simulink model "Controller"  (R2018b)
settings: configuration reference "control_config" (kept outside this file)
values from neighbouring files (symbols this model uses):
  CONTROL_EXPORT = Simulink.Parameter(CONTROL_EXPORT_VALUE)    [controller_model_init.m]
  CONTROL_PARAM = Simulink.Parameter(CONTROL_PARAM_VALUE)    [controller_model_init.m]
undefined symbols (not defined in the file or in its folder): actuator_cmd, CONTROL_CONST, DiscIntNeverNeededParam, timestamp
libraries: FMT_Model_Lib x5, simulink x1
settings Model: Creator=jc  LastModifiedBy=zouji
settings ConfigSetRef: SourceLocation=Base Workspace

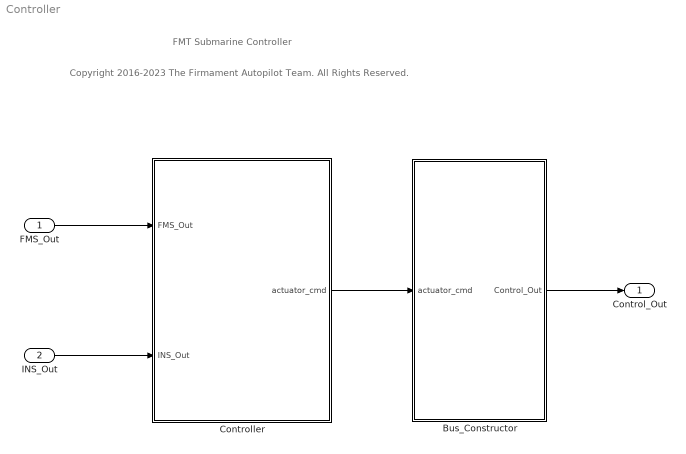
== system Controller ==
  note: Copyright 2016-2023 The Firmament Autopilot Team. All Rights Reserved.
  note: FMT Submarine Controller
  FMS_Out : Inport  OutDataTypeStr=Bus: FMS_Out_Bus
  INS_Out : Inport  Port=2  OutDataTypeStr=Bus: INS_Out_Bus
  Bus_Constructor : Subsystem
  Controller : Subsystem
  Control_Out : Outport  OutDataTypeStr=Bus: Control_Out_Bus
  wires:
  FMS_Out/1 -> Controller/1(FMS_Out)
  INS_Out/1 -> Controller/2(INS_Out)
  Controller/1(actuator_cmd) -> Bus_Constructor/1(actuator_cmd)
  Bus_Constructor/1(Control_Out) -> Control_Out/1

== system Controller/Bus_Constructor ==
  actuator_cmd : Inport
  Bus Assignment : BusAssignment  AssignedSignals=actuator_cmd,timestamp
  Constant : Constant  Value=0  OutDataTypeStr=Bus: Control_Out_Bus
  timestamp : Subsystem  mask{sample_time=CONTROL_EXPORT.period}
      mask prompts: sample_time "sample time (ms)"
  Control_Out : Outport
  wires:
  actuator_cmd/1 -> Bus Assignment/2
  Constant/1 -> Bus Assignment/1
  Bus Assignment/1 -> Control_Out/1
  timestamp/1(timestamp_ms) -> Bus Assignment/3

== system Controller/Controller ==
  FMS_Out : Inport
  INS_Out : Inport  Port=2
  Attitude_Controller : Subsystem
  Control_Allocation : Subsystem  Variant=on
      settings: GeneratePreprocessorConditionals=on
  Velocity_Controller : Subsystem
  actuator_cmd : Outport
  wires:
  Control_Allocation/1(actuator_cmd) -> actuator_cmd/1
  Attitude_Controller/1(torque_cmd_B) -> Control_Allocation/2(ang_acc_cmd)
  Velocity_Controller/1(force_cmd_B) -> Control_Allocation/3(line_acc_cmd)
  FMS_Out/1 -> Velocity_Controller/1(FMS_Out), Control_Allocation/1(FMS_Out), Attitude_Controller/1(FMS_Out)
  INS_Out/1 -> Velocity_Controller/2(INS_Out), Attitude_Controller/2(INS_Out)

== system Controller/Bus_Constructor/timestamp ==
  Constant : Constant  Value=sample_time
  Data Type Conversion : DataTypeConversion  OutDataTypeStr=uint32
  Discrete-Time Integrator : DiscreteIntegrator  IntegratorMethod=Accumulation: Forward Euler  SampleTime=-1  ICPrevOutput=DiscIntNeverNeededParam  ICPrevScaledInput=DiscIntNeverNeededParam
  timestamp_ms : Outport
  wires:
  Discrete-Time Integrator/1 -> Data Type Conversion/1
  Constant/1 -> Discrete-Time Integrator/1
  Data Type Conversion/1 -> timestamp_ms/1

== system Controller/Controller/Attitude_Controller ==
  FMS_Out : Inport
  INS_Out : Inport  Port=2
  Inner_Loop : Subsystem
  Outter_Loop : Subsystem
  Saturation1 : Saturate  UpperLimit=1  LowerLimit=-1
  torque_cmd_B : Outport
  wires:
  INS_Out/1 -> Inner_Loop/2(INS_Out), Outter_Loop/1(INS_Out)
  FMS_Out/1 -> Inner_Loop/3(FMS_Out), Outter_Loop/2(FMS_Out)
  Outter_Loop/1(rate_cmd_radPs) -> Inner_Loop/1(rate_cmd_radPs)
  Inner_Loop/1(rate_dot_cmd_B) -> Saturation1/1
  Saturation1/1 -> torque_cmd_B/1

== system Controller/Controller/Control_Allocation ==
  note: 1) Add Subsystem or Model blocks as valid variant choices.
      | 2) You cannot connect blocks at this level. At simulation, connectivity is automatically
      | determined, based on the active variant and port name matching.
  FMS_Out : Inport
  ang_acc_cmd : Inport  Port=2
  line_acc_cmd : Inport  Port=3
  Submarine_1 : Subsystem  TreatAsAtomicUnit=on  VariantControl=AIRFRAME==1
      mask Display: image('D:\ws\FMT\FMT-Model\figures\submarine_1.png');
  actuator_cmd : Outport

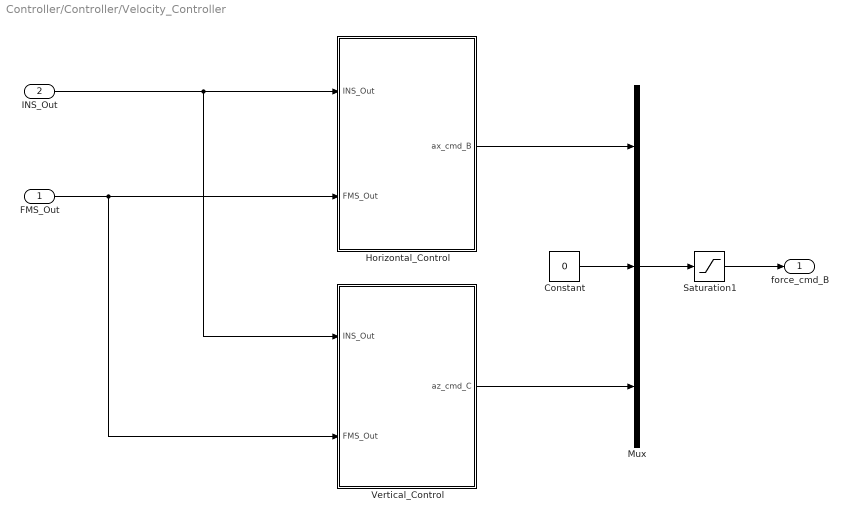
== system Controller/Controller/Velocity_Controller ==
  FMS_Out : Inport
  INS_Out : Inport  Port=2
  Constant : Constant  Value=0  OutDataTypeStr=single
  Horizontal_Control : Subsystem
  Mux : Mux  Inputs=3
  Saturation1 : Saturate  UpperLimit=1  LowerLimit=-1
  Vertical_Control : Subsystem
  force_cmd_B : Outport
  wires:
  FMS_Out/1 -> Vertical_Control/2(FMS_Out), Horizontal_Control/2(FMS_Out)
  Mux/1 -> Saturation1/1
  INS_Out/1 -> Vertical_Control/1(INS_Out), Horizontal_Control/1(INS_Out)
  Horizontal_Control/1(ax_cmd_B) -> Mux/1
  Vertical_Control/1(az_cmd_C) -> Mux/3
  Constant/1 -> Mux/2
  Saturation1/1 -> force_cmd_B/1

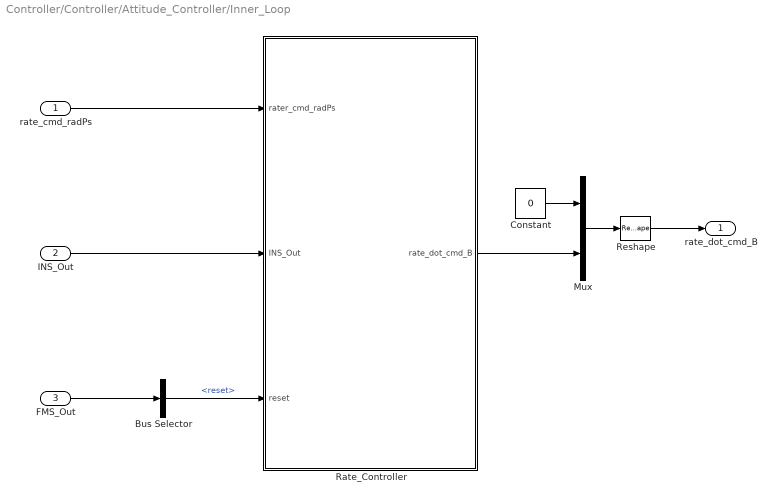
== system Controller/Controller/Attitude_Controller/Inner_Loop ==
  rate_cmd_radPs : Inport
  INS_Out : Inport  Port=2
  FMS_Out : Inport  Port=3
  Bus Selector : BusSelector  OutputSignals=reset
  Constant : Constant  Value=0  OutDataTypeStr=single
  Mux : Mux  Inputs=2
  Rate_Controller : Subsystem
  Reshape : Reshape  OutputDimensionality=Column vector (2-D)
  rate_dot_cmd_B : Outport
  wires:
  Rate_Controller/1(rate_dot_cmd_B) -> Mux/2
  Bus Selector/1 -> Rate_Controller/3(reset)  "<reset>"
  INS_Out/1 -> Rate_Controller/2(INS_Out)
  FMS_Out/1 -> Bus Selector/1
  Mux/1 -> Reshape/1
  Constant/1 -> Mux/1
  rate_cmd_radPs/1 -> Rate_Controller/1(rater_cmd_radPs)
  Reshape/1 -> rate_dot_cmd_B/1

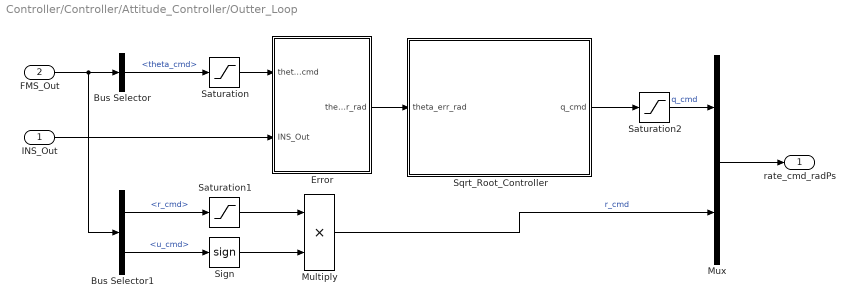
== system Controller/Controller/Attitude_Controller/Outter_Loop ==
  INS_Out : Inport
  FMS_Out : Inport  Port=2
  Bus Selector : BusSelector  OutputSignals=theta_cmd
  Bus Selector1 : BusSelector  OutputSignals=r_cmd,u_cmd
  Error : Subsystem
  Multiply : Product
  Mux : Mux  Inputs=2
  Saturation : Saturate  UpperLimit=CONTROL_PARAM.PITCH_CMD_LIM  LowerLimit=-CONTROL_PARAM.PITCH_CMD_LIM
  Saturation1 : Saturate  UpperLimit=CONTROL_PARAM.R_CMD_LIM  LowerLimit=-CONTROL_PARAM.R_CMD_LIM
  Saturation2 : Saturate  UpperLimit=CONTROL_PARAM.Q_CMD_LIM  LowerLimit=-CONTROL_PARAM.Q_CMD_LIM
  Sign : Signum
  Sqrt_Root_Controller : Subsystem
  rate_cmd_radPs : Outport
  wires:
  Bus Selector/1 -> Saturation/1  "<theta_cmd>"
  FMS_Out/1 -> Bus Selector1/1, Bus Selector/1
  Sqrt_Root_Controller/1(q_cmd) -> Saturation2/1
  Error/1(theta_err_rad) -> Sqrt_Root_Controller/1(theta_err_rad)
  INS_Out/1 -> Error/2(INS_Out)
  Saturation/1 -> Error/1(theta_cmd)
  Bus Selector1/1 -> Saturation1/1  "<r_cmd>"
  Mux/1 -> rate_cmd_radPs/1
  Saturation2/1 -> Mux/1  "q_cmd"
  Bus Selector1/2 -> Sign/1  "<u_cmd>"
  Saturation1/1 -> Multiply/1
  Sign/1 -> Multiply/2
  Multiply/1 -> Mux/2  "r_cmd"

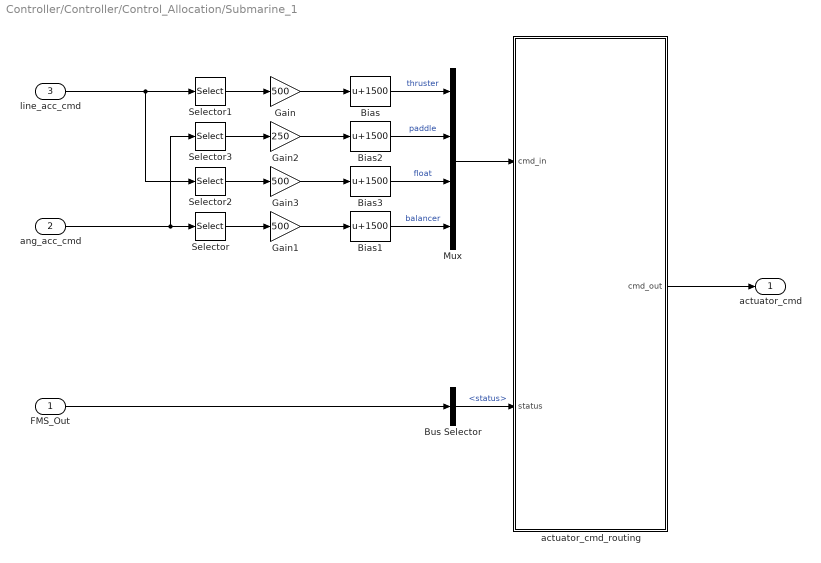
== system Controller/Controller/Control_Allocation/Submarine_1 ==
  FMS_Out : Inport
  ang_acc_cmd : Inport  Port=2
  line_acc_cmd : Inport  Port=3
  Bias{,1..3} (4 alike) : Bias  Bias=1500
  Bus Selector : BusSelector  OutputSignals=status
  Gain : Gain  Gain=500  OutDataTypeStr=uint16
  Gain1 : Gain  Gain=500  OutDataTypeStr=uint16
  Gain2 : Gain  Gain=250  OutDataTypeStr=uint16
  Gain3 : Gain  Gain=500  OutDataTypeStr=uint16
  Mux : Mux
  Selector : Selector  InputPortWidth=3  IndexOptions=Index vector (dialog)  Indices=2  OutputSizes=1
  Selector1 : Selector  InputPortWidth=3  IndexOptions=Index vector (dialog)  Indices=1  OutputSizes=1
  Selector2 : Selector  InputPortWidth=3  IndexOptions=Index vector (dialog)  Indices=3  OutputSizes=1
  Selector3 : Selector  InputPortWidth=3  IndexOptions=Index vector (dialog)  Indices=3  OutputSizes=1
  actuator_cmd_routing : Subsystem
  actuator_cmd : Outport
  wires:
  FMS_Out/1 -> Bus Selector/1
  actuator_cmd_routing/1(cmd_out) -> actuator_cmd/1
  Mux/1 -> actuator_cmd_routing/1(cmd_in)
  Bus Selector/1 -> actuator_cmd_routing/2(status)  "<status>"
  Gain/1 -> Bias/1
  Gain1/1 -> Bias1/1
  ang_acc_cmd/1 -> Selector3/1, Selector/1
  Bias/1 -> Mux/1  "thruster"
  Bias1/1 -> Mux/4  "balancer"
  Gain2/1 -> Bias2/1
  Gain3/1 -> Bias3/1
  Selector1/1 -> Gain/1
  Selector3/1 -> Gain2/1
  Selector2/1 -> Gain3/1
  Bias2/1 -> Mux/2  "paddle"
  Bias3/1 -> Mux/3  "float"
  Selector/1 -> Gain1/1
  line_acc_cmd/1 -> Selector1/1, Selector2/1

== system Controller/Controller/Velocity_Controller/Horizontal_Control ==
  INS_Out : Inport
  FMS_Out : Inport  Port=2
  Bus Selector : BusSelector  OutputSignals=reset
  Error : Subsystem
  PID_Controller : Subsystem
  ax_cmd_B : Outport
  wires:
  Error/1(u_err_B_mPs) -> PID_Controller/1(u_err_B_mPs)
  Bus Selector/1 -> PID_Controller/2(reset)  "<reset>"
  FMS_Out/1 -> Error/2(FMS_Out), Bus Selector/1
  PID_Controller/1(ax_cmd_B) -> ax_cmd_B/1
  INS_Out/1 -> Error/1(INS_Out)

== system Controller/Controller/Velocity_Controller/Vertical_Control ==
  INS_Out : Inport
  FMS_Out : Inport  Port=2
  Bus Selector : BusSelector  OutputSignals=reset
  Error : Subsystem
  PID_Controller : Subsystem
  az_cmd_C : Outport
  wires:
  PID_Controller/1(az_cmd) -> az_cmd_C/1
  Bus Selector/1 -> PID_Controller/2(reset)  "<reset>"
  Error/1(w_cmd_C_mPs) -> PID_Controller/1(w_cmd_C_mPs)
  INS_Out/1 -> Error/2(INS_Out)
  FMS_Out/1 -> Bus Selector/1, Error/1(FMS_Out)

== system Controller/Controller/Attitude_Controller/Inner_Loop/Rate_Controller ==
  rater_cmd_radPs : Inport
  INS_Out : Inport  Port=2
  reset : Inport  Port=3
  Error : Subsystem
  PID_Controller : Subsystem
  rate_dot_cmd_B : Outport
  wires:
  INS_Out/1 -> Error/2(INS_Out)
  Error/1(rate_err_radPs) -> PID_Controller/1(rate_err_C_mPs)
  rater_cmd_radPs/1 -> Error/1(rater_cmd_radPs)
  reset/1 -> PID_Controller/2(reset)
  PID_Controller/1(rate_dot_cmd_C) -> rate_dot_cmd_B/1

== system Controller/Controller/Attitude_Controller/Outter_Loop/Error ==
  theta_cmd : Inport
  INS_Out : Inport  Port=2
  Bus_Select : Subsystem
  Sum : Sum  Inputs=|+-
  theta_err_rad : Outport
  wires:
  theta_cmd/1 -> Sum/1  "theta_cmd_B_rad"
  Sum/1 -> theta_err_rad/1  "theta_error_B_rad"
  INS_Out/1 -> Bus_Select/1(INS_Out)
  Bus_Select/1(theta_est_B_rad) -> Sum/2  "theta_est_B_rad"

== system Controller/Controller/Attitude_Controller/Outter_Loop/Sqrt_Root_Controller ==
  theta_err_rad : Inport
  Constant2 : Constant  Value=CONTROL_PARAM.PITCH_P
  Sqrt_Root_Control : Subsystem  mask{dt=CONTROL_CONST.dt, second_ord_lim=9.5993}
      mask prompts: second_ord_lim "2nd-order lim"
  q_cmd : Outport
  wires:
  Sqrt_Root_Control/1(out) -> q_cmd/1
  theta_err_rad/1 -> Sqrt_Root_Control/1(error)
  Constant2/1 -> Sqrt_Root_Control/2(p)

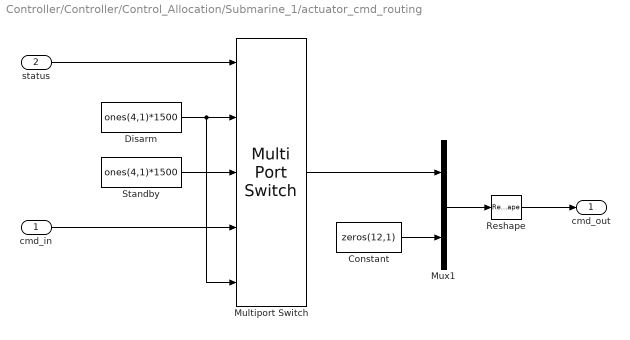
== system Controller/Controller/Control_Allocation/Submarine_1/actuator_cmd_routing ==
  cmd_in : Inport
  status : Inport  Port=2
  Constant : Constant  Value=zeros(12,1)  VectorParams1D=off  OutDataTypeStr=uint16
  Disarm : Constant  Value=ones(4,1)*1500  VectorParams1D=off  OutDataTypeStr=uint16
  Multiport Switch : MultiPortSwitch  DataPortForDefault=Additional data port  DiagnosticForDefault=None
  Mux1 : Mux  Inputs=2
  Reshape : Reshape  OutputDimensionality=Customize  OutputDimensions=[16,1]
  Standby : Constant  Value=ones(4,1)*1500  VectorParams1D=off  OutDataTypeStr=uint16
  cmd_out : Outport
  wires:
  Disarm/1 -> Multiport Switch/5, Multiport Switch/2
  Reshape/1 -> cmd_out/1
  Constant/1 -> Mux1/2
  Standby/1 -> Multiport Switch/3
  Mux1/1 -> Reshape/1
  status/1 -> Multiport Switch/1
  Multiport Switch/1 -> Mux1/1
  cmd_in/1 -> Multiport Switch/4

== system Controller/Controller/Velocity_Controller/Horizontal_Control/Error ==
  INS_Out : Inport
  FMS_Out : Inport  Port=2
  Bus Selector : BusSelector  OutputSignals=u_cmd
  Bus_Select : Subsystem
  Sum : Sum  Inputs=|+-
  u_err_B_mPs : Outport
  wires:
  Sum/1 -> u_err_B_mPs/1  "u_error_B_mPs"
  FMS_Out/1 -> Bus Selector/1
  INS_Out/1 -> Bus_Select/1(INS_Out)
  Bus_Select/1(u_est_B_mPs) -> Sum/2  "u_est_B_mPs"
  Bus Selector/1 -> Sum/1  "<u_cmd>"

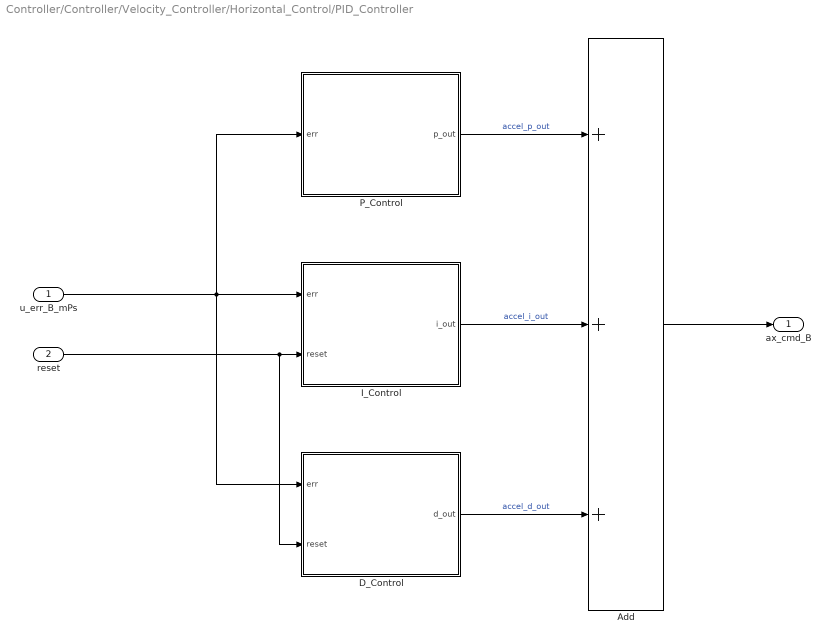
== system Controller/Controller/Velocity_Controller/Horizontal_Control/PID_Controller ==
  u_err_B_mPs : Inport
  reset : Inport  Port=2
  Add : Sum  Inputs=+++
  D_Control : Subsystem  mask{kd=CONTROL_PARAM.VEL_X_D, max_d=CONTROL_PARAM.VEL_X_D_MAX, min_d=CONTROL_PARAM.VEL_X_D_MIN}
  I_Control : Subsystem  mask{ki=CONTROL_PARAM.VEL_X_I, max_i=CONTROL_PARAM.VEL_X_I_MAX, min_i=CONTROL_PARAM.VEL_X_I_MIN}
  P_Control : Subsystem  mask{kp=CONTROL_PARAM.VEL_X_P}
  ax_cmd_B : Outport
  wires:
  u_err_B_mPs/1 -> P_Control/1(err), I_Control/1(err), D_Control/1(err)
  reset/1 -> I_Control/2(reset), D_Control/2(reset)
  P_Control/1(p_out) -> Add/1  "accel_p_out"
  I_Control/1(i_out) -> Add/2  "accel_i_out"
  D_Control/1(d_out) -> Add/3  "accel_d_out"
  Add/1 -> ax_cmd_B/1

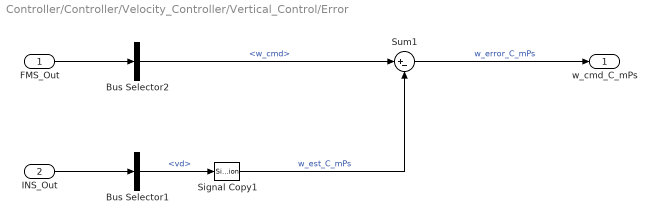
== system Controller/Controller/Velocity_Controller/Vertical_Control/Error ==
  FMS_Out : Inport
  INS_Out : Inport  Port=2
  Bus Selector1 : BusSelector  OutputSignals=vd
  Bus Selector2 : BusSelector  OutputSignals=w_cmd
  Signal Copy1 : SignalConversion  OverrideOpt=off
  Sum1 : Sum  Inputs=|+-
  w_cmd_C_mPs : Outport
  wires:
  INS_Out/1 -> Bus Selector1/1
  Bus Selector2/1 -> Sum1/1  "<w_cmd>"
  Bus Selector1/1 -> Signal Copy1/1  "<vd>"
  Sum1/1 -> w_cmd_C_mPs/1  "w_error_C_mPs"
  FMS_Out/1 -> Bus Selector2/1
  Signal Copy1/1 -> Sum1/2  "w_est_C_mPs"

== system Controller/Controller/Velocity_Controller/Vertical_Control/PID_Controller ==
  w_cmd_C_mPs : Inport
  reset : Inport  Port=2
  Add : Sum  Inputs=+++
  D_Control : Subsystem  mask{kd=CONTROL_PARAM.VEL_Z_D, max_d=CONTROL_PARAM.VEL_Z_D_MAX, min_d=CONTROL_PARAM.VEL_Z_D_MIN}
  I_Control : Subsystem  mask{ki=CONTROL_PARAM.VEL_Z_I, max_i=CONTROL_PARAM.VEL_Z_I_MAX, min_i=CONTROL_PARAM.VEL_Z_I_MIN}
  P_Control : Subsystem  mask{kp=CONTROL_PARAM.VEL_Z_P}
  az_cmd : Outport
  wires:
  P_Control/1(p_out) -> Add/1  "thrust_p_out"
  I_Control/1(i_out) -> Add/2  "thrust_i_out"
  Add/1 -> az_cmd/1
  w_cmd_C_mPs/1 -> D_Control/1(err), I_Control/1(err), P_Control/1(err)
  D_Control/1(d_out) -> Add/3  "thrust_d_out"
  reset/1 -> I_Control/2(reset), D_Control/2(reset)

== system Controller/Controller/Attitude_Controller/Inner_Loop/Rate_Controller/Error ==
  rater_cmd_radPs : Inport
  INS_Out : Inport  Port=2
  Bus_Select : Subsystem
  First Order LPF : FMT_Model_Lib/Filter/First Order LPF  fc=30
      settings: SourceProductName=FMT Toolbox
  Sum : Sum  Inputs=|+-
  rate_err_radPs : Outport
  wires:
  Sum/1 -> First Order LPF/1  "rate_error_B_radPs"
  rater_cmd_radPs/1 -> Sum/1  "rate_cmd_B_radPs"
  INS_Out/1 -> Bus_Select/1(INS_Out)
  Bus_Select/1(rate_est_radPs) -> Sum/2  "rate_est_B_radPs"
  First Order LPF/1 -> rate_err_radPs/1

== system Controller/Controller/Attitude_Controller/Inner_Loop/Rate_Controller/PID_Controller ==
  rate_err_C_mPs : Inport
  reset : Inport  Port=2
  Add : Sum  Inputs=+++
  D_Control : Subsystem  mask{q_kd=CONTROL_PARAM.PITCH_RATE_D, r_kd=CONTROL_PARAM.YAW_RATE_D, max_d=CONTROL_PARAM.RATE_D_MAX, min_d=CONTROL_PARAM.RATE_D_MIN}
  I_Control : Subsystem  mask{q_ki=CONTROL_PARAM.PITCH_RATE_I, r_ki=CONTROL_PARAM.YAW_RATE_I, max_i=CONTROL_PARAM.RATE_I_MAX, min_i=CONTROL_PARAM.RATE_I_MIN}
  P_Control : Subsystem  mask{q_kp=CONTROL_PARAM.PITCH_RATE_P, r_kp=CONTROL_PARAM.YAW_RATE_P}
  rate_dot_cmd_C : Outport
  wires:
  rate_err_C_mPs/1 -> P_Control/1(err), I_Control/1(err), D_Control/1(err)
  reset/1 -> I_Control/2(reset), D_Control/2(reset)
  P_Control/1(p_out) -> Add/1  "accel_p_out"
  I_Control/1(i_out) -> Add/2  "accel_i_out"
  D_Control/1(d_out) -> Add/3  "accel_d_out"
  Add/1 -> rate_dot_cmd_C/1

== system Controller/Controller/Attitude_Controller/Outter_Loop/Error/Bus_Select ==
  INS_Out : Inport
  Bus Selector1 : BusSelector  OutputSignals=theta
  theta_est_B_rad : Outport
  wires:
  INS_Out/1 -> Bus Selector1/1
  Bus Selector1/1 -> theta_est_B_rad/1  "<theta>"

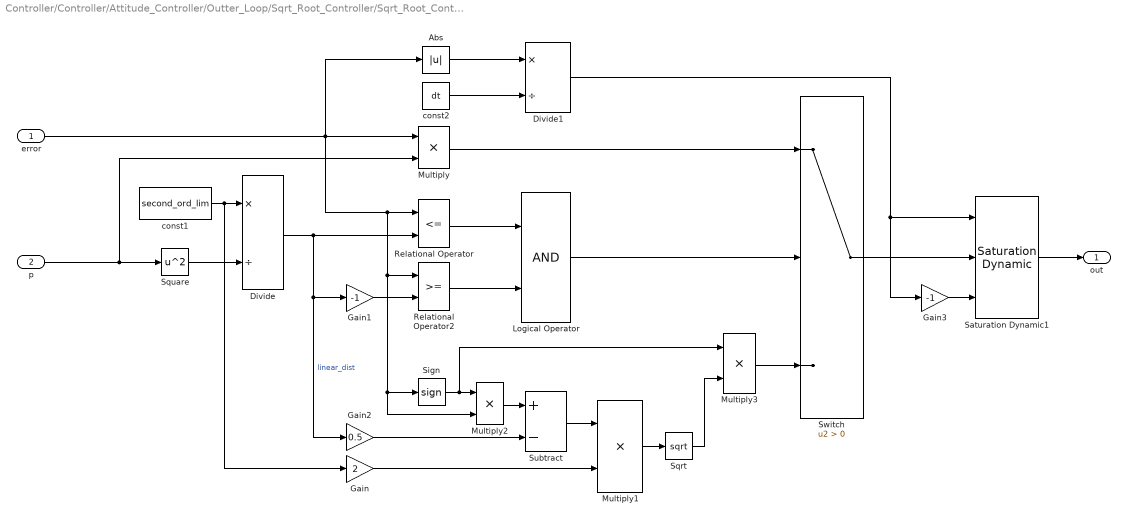
== system Controller/Controller/Attitude_Controller/Outter_Loop/Sqrt_Root_Controller/Sqrt_Root_Control ==
  error : Inport
  p : Inport  Port=2
  Abs : Abs
  Divide : Product  Inputs=*/
  Divide1 : Product  Inputs=*/
  Gain : Gain  Gain=2  OutDataTypeStr=Inherit: Same as input
  Gain1 : Gain  Gain=-1  OutDataTypeStr=Inherit: Same as input
  Gain2 : Gain  Gain=0.5  OutDataTypeStr=Inherit: Same as input
  Gain3 : Gain  Gain=-1  OutDataTypeStr=Inherit: Same as input
  Logical Operator : Logic  AllPortsSameDT=off  OutDataTypeStr=boolean
  Multiply{,1..3} (4 alike) : Product
  Relational Operator : RelationalOperator  Operator=<=  OutDataTypeStr=boolean  RndMeth=Simplest
  Relational Operator2 : RelationalOperator  OutDataTypeStr=boolean  RndMeth=Simplest
  Saturation Dynamic1 : simulink/Discontinuities/Saturation Dynamic  OutMin=[]  OutMax=[]  OutDataTypeStr=Inherit: Same as second input  OutDataType=fixdt(1, 16)  OutScaling=2^-10  DoSatur=off
  Sign : Signum
  Sqrt : Sqrt  SaturateOnIntegerOverflow=on
  Square : Math  Operator=square  SaturateOnIntegerOverflow=on
  Subtract : Sum  Inputs=+-
  Switch : Switch  Criteria=u2 > Threshold
  const1 : Constant  Value=second_ord_lim  OutDataTypeStr=single
  const2 : Constant  Value=dt  OutDataTypeStr=single
  out : Outport
  wires:
  p/1 -> Multiply/2, Square/1
  const1/1 -> Gain/1, Divide/1
  Square/1 -> Divide/2
  Divide/1 -> Gain2/1, Gain1/1, Relational Operator/2  "linear_dist"
  error/1 -> Abs/1, Multiply/1, Multiply2/2, Sign/1, Relational Operator2/1, Relational Operator/1
  Relational Operator/1 -> Logical Operator/1
  Multiply/1 -> Switch/1
  Switch/1 -> Saturation Dynamic1/2
  Multiply3/1 -> Switch/3
  Gain/1 -> Multiply1/2
  Gain1/1 -> Relational Operator2/2
  Relational Operator2/1 -> Logical Operator/2
  Logical Operator/1 -> Switch/2
  Gain2/1 -> Subtract/2
  Sign/1 -> Multiply3/1, Multiply2/1
  Multiply2/1 -> Subtract/1
  Subtract/1 -> Multiply1/1
  Multiply1/1 -> Sqrt/1
  Sqrt/1 -> Multiply3/2
  Saturation Dynamic1/1 -> out/1
  Abs/1 -> Divide1/1
  const2/1 -> Divide1/2
  Divide1/1 -> Gain3/1, Saturation Dynamic1/1
  Gain3/1 -> Saturation Dynamic1/3

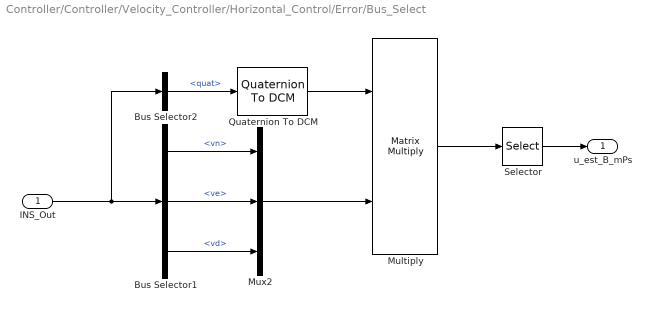
== system Controller/Controller/Velocity_Controller/Horizontal_Control/Error/Bus_Select ==
  INS_Out : Inport
  Bus Selector1 : BusSelector  OutputSignals=vn,ve,vd
  Bus Selector2 : BusSelector  OutputSignals=quat
  Multiply : Product  Multiplication=Matrix(*)
  Mux2 : Mux  Inputs=3
  Quaternion To DCM : FMT_Model_Lib/Quaternion/Quaternion To DCM
      settings: SourceProductName=FMT Toolbox
  Selector : Selector  InputPortWidth=3  IndexOptions=Index vector (dialog)  Indices=1  OutputSizes=1
  u_est_B_mPs : Outport
  wires:
  Quaternion To DCM/1 -> Multiply/1
  Bus Selector2/1 -> Quaternion To DCM/1  "<quat>"
  Mux2/1 -> Multiply/2
  Bus Selector1/2 -> Mux2/2  "<ve>"
  Bus Selector1/1 -> Mux2/1  "<vn>"
  INS_Out/1 -> Bus Selector2/1, Bus Selector1/1
  Multiply/1 -> Selector/1
  Selector/1 -> u_est_B_mPs/1
  Bus Selector1/3 -> Mux2/3  "<vd>"

== system Controller/Controller/Velocity_Controller/Horizontal_Control/PID_Controller/D_Control ==
  err : Inport
  reset : Inport  Port=2
  DT Filter : FMT_Model_Lib/Filter/DT Filter  fc=10
      settings: SourceProductName=FMT Toolbox
  Multiply : Product  OutDataTypeStr=Inherit: Same as first input
  Saturation : Saturate  UpperLimit=max_d  LowerLimit=min_d
  kd : Constant  Value=kd  OutDataTypeStr=single
  d_out : Outport
  wires:
  err/1 -> DT Filter/1
  kd/1 -> Multiply/1
  Multiply/1 -> Saturation/1
  Saturation/1 -> d_out/1
  reset/1 -> DT Filter/2
  DT Filter/1 -> Multiply/2

== system Controller/Controller/Velocity_Controller/Horizontal_Control/PID_Controller/I_Control ==
  err : Inport
  reset : Inport  Port=2
  Constant : Constant  Value=0  OutDataTypeStr=single
  Discrete-Time Integrator : DiscreteIntegrator  ExternalReset=level  InitialConditionSource=external  SampleTime=-1  LimitOutput=on  UpperSaturationLimit=max_i  LowerSaturationLimit=min_i  ICPrevOutput=DiscIntNeverNeededParam  ICPrevScaledInput=DiscIntNeverNeededParam
  Multiply : Product  OutDataTypeStr=Inherit: Same as first input
  ki : Constant  Value=ki  OutDataTypeStr=single
  i_out : Outport
  wires:
  err/1 -> Multiply/2
  Multiply/1 -> Discrete-Time Integrator/1
  reset/1 -> Discrete-Time Integrator/2
  Constant/1 -> Discrete-Time Integrator/3
  Discrete-Time Integrator/1 -> i_out/1
  ki/1 -> Multiply/1

== system Controller/Controller/Velocity_Controller/Horizontal_Control/PID_Controller/P_Control ==
  err : Inport
  Multiply : Product  OutDataTypeStr=Inherit: Same as first input
  kp : Constant  Value=kp  OutDataTypeStr=single
  p_out : Outport
  wires:
  err/1 -> Multiply/2
  kp/1 -> Multiply/1
  Multiply/1 -> p_out/1

== system Controller/Controller/Velocity_Controller/Vertical_Control/PID_Controller/D_Control ==
  err : Inport
  reset : Inport  Port=2
  DT Filter : FMT_Model_Lib/Filter/DT Filter  fc=10
      settings: SourceProductName=FMT Toolbox
  Multiply : Product  OutDataTypeStr=Inherit: Same as first input
  Saturation : Saturate  UpperLimit=max_d  LowerLimit=min_d
  kd : Constant  Value=kd  OutDataTypeStr=single
  d_out : Outport
  wires:
  err/1 -> DT Filter/1
  kd/1 -> Multiply/1
  Multiply/1 -> Saturation/1
  Saturation/1 -> d_out/1
  reset/1 -> DT Filter/2
  DT Filter/1 -> Multiply/2

== system Controller/Controller/Velocity_Controller/Vertical_Control/PID_Controller/I_Control ==
  err : Inport
  reset : Inport  Port=2
  Constant : Constant  Value=min_i  OutDataTypeStr=single
  Discrete-Time Integrator : DiscreteIntegrator  ExternalReset=level  InitialConditionSource=external  SampleTime=-1  LimitOutput=on  UpperSaturationLimit=max_i  LowerSaturationLimit=min_i  ICPrevOutput=DiscIntNeverNeededParam  ICPrevScaledInput=DiscIntNeverNeededParam
  Multiply : Product  OutDataTypeStr=Inherit: Same as first input
  ki : Constant  Value=ki  OutDataTypeStr=single
  i_out : Outport
  wires:
  err/1 -> Multiply/2
  Multiply/1 -> Discrete-Time Integrator/1
  reset/1 -> Discrete-Time Integrator/2
  Constant/1 -> Discrete-Time Integrator/3
  Discrete-Time Integrator/1 -> i_out/1
  ki/1 -> Multiply/1

== system Controller/Controller/Velocity_Controller/Vertical_Control/PID_Controller/P_Control ==
  err : Inport
  Multiply : Product  OutDataTypeStr=Inherit: Same as first input
  kp : Constant  Value=kp  OutDataTypeStr=single
  p_out : Outport
  wires:
  err/1 -> Multiply/2
  kp/1 -> Multiply/1
  Multiply/1 -> p_out/1

== system Controller/Controller/Attitude_Controller/Inner_Loop/Rate_Controller/Error/Bus_Select ==
  INS_Out : Inport
  Bus Selector1 : BusSelector  OutputSignals=q,r
  Mux : Mux  Inputs=2
  rate_est_radPs : Outport
  wires:
  INS_Out/1 -> Bus Selector1/1
  Bus Selector1/1 -> Mux/1  "<q>"
  Bus Selector1/2 -> Mux/2  "<r>"
  Mux/1 -> rate_est_radPs/1

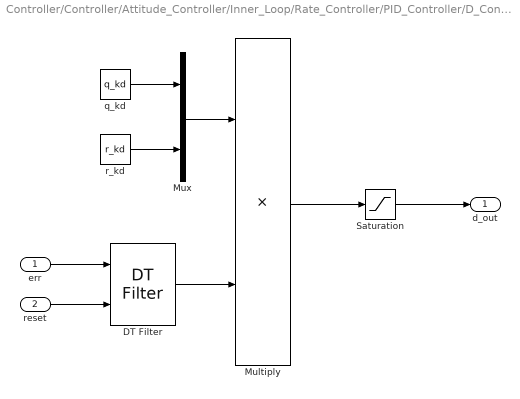
== system Controller/Controller/Attitude_Controller/Inner_Loop/Rate_Controller/PID_Controller/D_Control ==
  err : Inport
  reset : Inport  Port=2
  DT Filter : FMT_Model_Lib/Filter/DT Filter  fc=10
      settings: SourceProductName=FMT Toolbox
  Multiply : Product  OutDataTypeStr=Inherit: Same as first input
  Mux : Mux  Inputs=2
  Saturation : Saturate  UpperLimit=max_d  LowerLimit=min_d
  q_kd : Constant  Value=q_kd  OutDataTypeStr=single
  r_kd : Constant  Value=r_kd  OutDataTypeStr=single
  d_out : Outport
  wires:
  err/1 -> DT Filter/1
  Multiply/1 -> Saturation/1
  Saturation/1 -> d_out/1
  reset/1 -> DT Filter/2
  DT Filter/1 -> Multiply/2
  Mux/1 -> Multiply/1
  q_kd/1 -> Mux/1
  r_kd/1 -> Mux/2

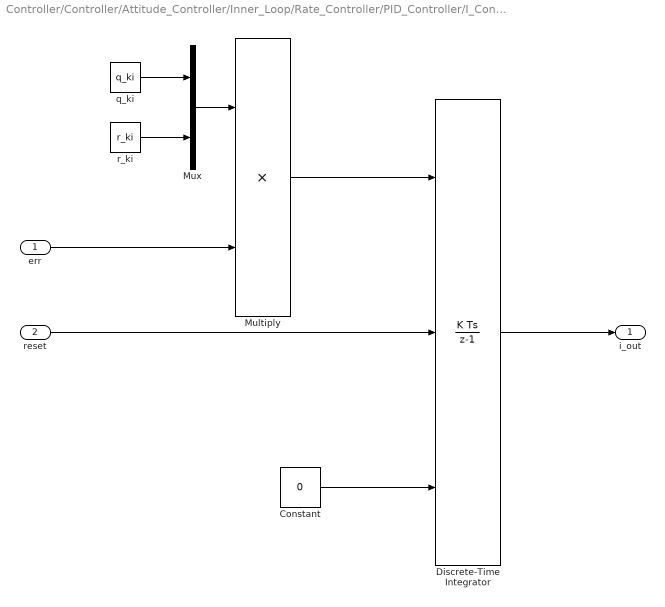
== system Controller/Controller/Attitude_Controller/Inner_Loop/Rate_Controller/PID_Controller/I_Control ==
  err : Inport
  reset : Inport  Port=2
  Constant : Constant  Value=0  OutDataTypeStr=single
  Discrete-Time Integrator : DiscreteIntegrator  ExternalReset=level  InitialConditionSource=external  SampleTime=-1  LimitOutput=on  UpperSaturationLimit=max_i  LowerSaturationLimit=min_i  ICPrevOutput=DiscIntNeverNeededParam  ICPrevScaledInput=DiscIntNeverNeededParam
  Multiply : Product  OutDataTypeStr=Inherit: Same as first input
  Mux : Mux  Inputs=2
  q_ki : Constant  Value=q_ki  OutDataTypeStr=single
  r_ki : Constant  Value=r_ki  OutDataTypeStr=single
  i_out : Outport
  wires:
  err/1 -> Multiply/2
  Multiply/1 -> Discrete-Time Integrator/1
  reset/1 -> Discrete-Time Integrator/2
  Constant/1 -> Discrete-Time Integrator/3
  Discrete-Time Integrator/1 -> i_out/1
  Mux/1 -> Multiply/1
  q_ki/1 -> Mux/1
  r_ki/1 -> Mux/2

== system Controller/Controller/Attitude_Controller/Inner_Loop/Rate_Controller/PID_Controller/P_Control ==
  err : Inport
  Multiply : Product  OutDataTypeStr=Inherit: Same as first input
  Mux : Mux  Inputs=2
  q_kp : Constant  Value=q_kp  OutDataTypeStr=single
  r_kp : Constant  Value=r_kp  OutDataTypeStr=single
  p_out : Outport
  wires:
  err/1 -> Multiply/2
  Multiply/1 -> p_out/1
  Mux/1 -> Multiply/1
  q_kp/1 -> Mux/1
  r_kp/1 -> Mux/2
